simulink model "native_M10_payload5kg_pose_hold_r2"  (R2026b)
settings: Solver=ode4  StopTime=35  FixedStep=2.5e-05  MaxStep=0.001  RelTol=1e-5
InitFcn:
  | addpath(fileparts(get_param(bdroot,'FileName')));
values from neighbouring files (symbols this model uses):
  s = block.Dwork(1).Data    [native_M10_payload5kg_pose_hold_r2_controller.m]
undefined symbols (not defined in the file or in its folder): X, Y, Z
libraries: sm_lib x42, nesl_utility x20
(part 1 of 2)
settings Model: Creator=lelfs  LastModifiedBy=lelfs
settings DataIOCC: LimitDataPoints=on  MaxDataPoints=10000
settings OptimizationCC: LifeSpan=inf  ReuseModelBlockBuffer=off
settings DebuggingCC: AllowSymbolicDim=off  ArithmeticOperatorsInVariantConditions=warning  SFExecutionAtInitializationDiag=none  SFNoUnconditionalDefaultTransitionDiag=warning  SFUnexpectedBacktrackingDiag=warning  SubsystemReferenceDiagnosticForUnitTest=warning
settings SFSimCC: CustomCodeUndefinedFunction=UseInterfaceOnly  SimUseLocalCustomCode=off
settings RTWCC: DLArmComputeVersion=19.05  RTWUseLocalCustomCode=off
settings CodeAppCC: StateflowObjectComments=on
settings GRTTargetCC: TargetLangStandard=C89/C90 (ANSI)
settings ConfigComp: CovExternalEMLEnable=off  CovSFcnEnable=off  CovSaveCumulativeToWorkspaceVar=on  CovSaveSingleToWorkspaceVar=on
settings SimscapeCC: SimscapeLogLimitData=off  SimscapeUseEnergyAccounting=off
settings ExplorerConfigSet: SimMechanicsOpenEditorOnUpdate=off

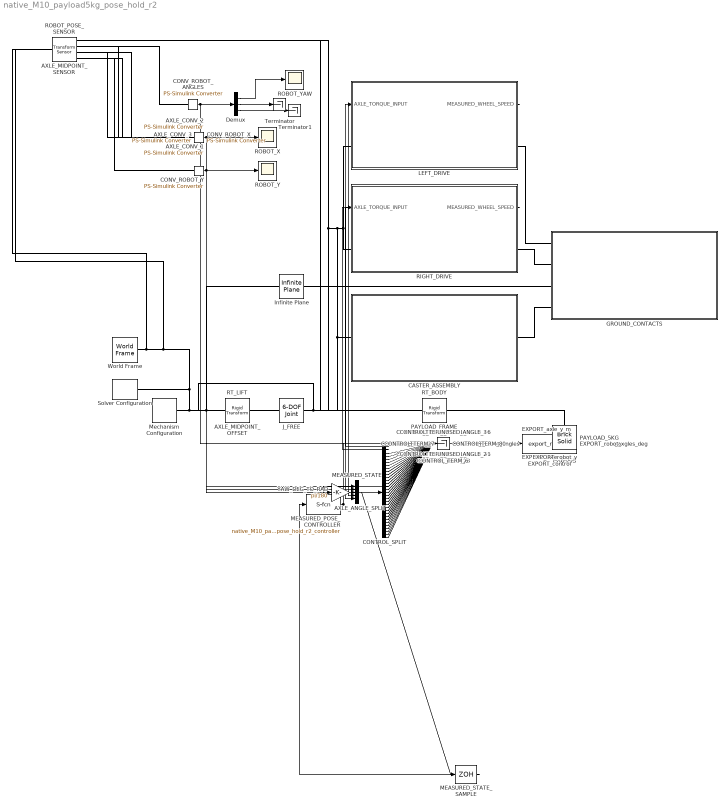
== system native_M10_payload5kg_pose_hold_r2 ==
  AXLE_ANGLE_SPLIT : Demux  Outputs=3
  AXLE_CONV_1 : nesl_utility/PS-Simulink Converter  PhysicalDomain=network_engine_domain  SubClassName=ps_output  LeftPortType=input  RightPortType=output  PseudoPeriodic=off  Frequencies=[]  VectorFormat=inherit  Unit=m  AffineConversion=off
  AXLE_CONV_2 : nesl_utility/PS-Simulink Converter  PhysicalDomain=network_engine_domain  SubClassName=ps_output  LeftPortType=input  RightPortType=output  PseudoPeriodic=off  Frequencies=[]  VectorFormat=inherit  Unit=m  AffineConversion=off
  AXLE_CONV_3 : nesl_utility/PS-Simulink Converter  PhysicalDomain=network_engine_domain  SubClassName=ps_output  LeftPortType=input  RightPortType=output  PseudoPeriodic=off  Frequencies=[]  VectorFormat=inherit  Unit=deg  AffineConversion=off
  AXLE_MIDPOINT_OFFSET : sm_lib/Frames and Transforms/Rigid Transform  RotationMethod=None  FollAlignAxisA=+X  BaseAlignAxisA=+Y  FollAlignAxisB=+Y  BaseAlignAxisB=+Z  RotationStandardAxis=+Z  RotationAngle=0  RotationAngleUnits=deg  RotationArbitraryAxis=[0 0 1]  RotationSequenceAxes=FollowerAxes  RotationSequence=XYX  RotationSequenceAngles=[0 0 0]  RotationSequenceAnglesUnits=deg  RotationMatrix=[1 0 0;0 1 0;0 0 1]  Quaternion=[1 0 0 0]  TranslationMethod=Cartesian  TranslationCartesianOffset=[0 0 0.075]  TranslationCartesianOffsetUnits=m  TranslationStandardAxis=+Z  TranslationStandardOffset=0  TranslationStandardOffsetUnits=m  TranslationROffset=0  TranslationROffsetUnits=m  TranslationThetaOffset=0  TranslationThetaOffsetUnits=deg  TranslationZOffset=0  TranslationZOffsetUnits=m
  AXLE_MIDPOINT_SENSOR : sm_lib/Frames and Transforms/Transform Sensor  ObservationFrame=World  ExpressedInFrame=World  RotationSequence=ZYX  SenseAngle=off  SenseAxis=off  SenseQ=off  SenseR=off  SenseRotationSequence=on  SenseOmegaX=off  SenseOmegaY=off  SenseOmegaZ=off  SenseOmega=off  SenseQDot=off  SenseRDot=off  SenseRotationSequenceDot=off  SenseAlphaX=off  SenseAlphaY=off  SenseAlphaZ=off  SenseAlpha=off  SenseQDDot=off  SenseRDDot=off  SenseX=on  SenseY=on  SenseZ=off  SenseXYZ=off  SenseRad=off  SenseAzim=off  SenseDist=off  SenseInc=off  SenseXDot=off  SenseYDot=off  SenseZDot=off  SenseXYZDot=off  SenseRadDot=off  SenseAzimDot=off  SenseDistDot=off  SenseIncDot=off  SenseXDDot=off  SenseYDDot=off  SenseZDDot=off  SenseXYZDDot=off  SenseRadDDot=off  SenseAzimDDot=off  SenseDistDDot=off  SenseIncDDot=off
  CASTER_ASSEMBLY : Subsystem
  CHASSIS : sm_lib/Body Elements/Brick Solid  BrickDimensions=[0.50 0.32 0.08]  BrickDimensionsUnits=m  ExportEntireGeometry=off  InertiaType=CalculateFromGeometry  BasedOnType=Mass  Density=1000  DensityUnits=kg/m^3  Mass=15.2  MassUnits=kg  CenterOfMass=[0 0 0]  CenterOfMassUnits=m  MomentsOfInertia=[1 1 1]  MomentsOfInertiaUnits=kg*m^2  ProductsOfInertia=[0 0 0]  ProductsOfInertiaUnits=kg*m^2  GraphicType=FromGeometry  MarkerShape=Sphere  MarkerSize=10  GraphicVisPropType=SimpleVisualProperties  GraphicDiffuseColor=[0.5 0.5 0.5]  GraphicOpacity=1.0  GraphicSpecularColor=[0.5 0.5 0.5 1.0]  GraphicAmbientColor=[0.15 0.15 0.15 1.0]  GraphicEmissiveColor=[0.0 0.0 0.0 1.0]  GraphicShininess=75  DoExposeReferenceFrame=on  SerializedFrames=<Frames/>
  CONTROL_SPLIT : Demux  Outputs=31
  CONTROL_TERM_{3..31} (29 alike) : Terminator
  CONV_ROBOT_ANGLES : nesl_utility/PS-Simulink Converter  PhysicalDomain=network_engine_domain  SubClassName=ps_output  LeftPortType=input  RightPortType=output  PseudoPeriodic=off  Frequencies=[]  VectorFormat=inherit  Unit=deg  AffineConversion=off
  CONV_ROBOT_X : nesl_utility/PS-Simulink Converter  PhysicalDomain=network_engine_domain  SubClassName=ps_output  LeftPortType=input  RightPortType=output  PseudoPeriodic=off  Frequencies=[]  VectorFormat=inherit  Unit=m  AffineConversion=off
  CONV_ROBOT_Y : nesl_utility/PS-Simulink Converter  PhysicalDomain=network_engine_domain  SubClassName=ps_output  LeftPortType=input  RightPortType=output  PseudoPeriodic=off  Frequencies=[]  VectorFormat=inherit  Unit=m  AffineConversion=off
  Demux : Demux  Outputs=3
  EXPORT_axle_angles_deg : ToWorkspace  VariableName=export_axle_angles_deg  SaveFormat=Timeseries  SampleTime=0.001
  EXPORT_axle_x_m : ToWorkspace  VariableName=export_axle_x_m  SaveFormat=Timeseries  SampleTime=0.001
  EXPORT_axle_y_m : ToWorkspace  VariableName=export_axle_y_m  SaveFormat=Timeseries  SampleTime=0.001
  EXPORT_control : ToWorkspace  VariableName=export_control  SaveFormat=Timeseries  SampleTime=0.001
  EXPORT_robot_angles : ToWorkspace  VariableName=export_robot_angles  SaveFormat=Timeseries  SampleTime=0.001
  EXPORT_robot_x : ToWorkspace  VariableName=export_robot_x  SaveFormat=Timeseries  SampleTime=0.001
  EXPORT_robot_y : ToWorkspace  VariableName=export_robot_y  SaveFormat=Timeseries  SampleTime=0.001
  GROUND_CONTACTS : Subsystem
  Infinite Plane : sm_lib/Curves and Surfaces/Infinite Plane  GraphicType=Rectangle  GraphicPlaneWidth=3  GraphicPlaneWidthUnits=m  GraphicPlaneHeight=3  GraphicPlaneHeightUnits=m  GraphicVisPropType=SimpleVisualProperties  GraphicDiffuseColor=[0.5 0.5 0.5]  GraphicOpacity=1  GraphicSpecularColor=[0.5 0.5 0.5 1.0]  GraphicAmbientColor=[0.15 0.15 0.15 1.0]  GraphicEmissiveColor=[0.0 0.0 0.0 1.0]  GraphicShininess=75
  J_FREE : sm_lib/Joints/6-DOF Joint  JointMode=Normal  CompositeWrenchDir=FollowerOnBase  CompositeWrenchFrame=BaseFrame  SenseConstraintForce=off  SenseConstraintTorque=off  SenseTotalForce=off  SenseTotalTorque=off  PxPositionTargetSpecify=on  PxPositionTargetPriority=High  PxPositionTargetValue=0  PxPositionTargetValueUnits=m  PxVelocityTargetSpecify=on  PxVelocityTargetPriority=High  PxVelocityTargetValue=0  PxVelocityTargetValueUnits=m/s  PxEquilibriumPosition=0  PxEquilibriumPositionUnits=m  PxSpringStiffness=0  PxSpringStiffnessUnits=N/m  PxDampingCoefficient=0  PxDampingCoefficientUnits=N/(m/s)  PxLowerLimitSpecify=off  PxLowerLimitBound=-1  PxLowerLimitBoundUnits=m  PxLowerLimitStiffness=1e6  PxLowerLimitStiffnessUnits=N/m  PxLowerLimitDamping=1e3  PxLowerLimitDampingUnits=N/(m/s)  PxLowerLimitTransitionRegionWidth=1e-4  PxLowerLimitTransitionRegionWidthUnits=m  PxUpperLimitSpecify=off  PxUpperLimitBound=1  PxUpperLimitBoundUnits=m  PxUpperLimitStiffness=1e6  PxUpperLimitStiffnessUnits=N/m  PxUpperLimitDamping=1e3  PxUpperLimitDampingUnits=N/(m/s)  PxUpperLimitTransitionRegionWidth=1e-4  PxUpperLimitTransitionRegionWidthUnits=m  PxTorqueActuationMode=NoTorque  PxMotionActuationMode=ComputedMotion  PxSensePosition=off  PxSenseVelocity=off  PxSenseAcceleration=off  PxSenseTorqueForce=off  PxSenseLowerLimitTorqueForce=off  PxSenseUpperLimitTorqueForce=off  PyPositionTargetSpecify=on  PyPositionTargetPriority=High  PyPositionTargetValue=0  PyPositionTargetValueUnits=m  PyVelocityTargetSpecify=on  PyVelocityTargetPriority=High  PyVelocityTargetValue=0  PyVelocityTargetValueUnits=m/s  PyEquilibriumPosition=0  PyEquilibriumPositionUnits=m  PySpringStiffness=0  PySpringStiffnessUnits=N/m  PyDampingCoefficient=0  PyDampingCoefficientUnits=N/(m/s)  PyLowerLimitSpecify=off  PyLowerLimitBound=-1  PyLowerLimitBoundUnits=m  PyLowerLimitStiffness=1e6  PyLowerLimitStiffnessUnits=N/m  PyLowerLimitDamping=1e3  PyLowerLimitDampingUnits=N/(m/s)  PyLowerLimitTransitionRegionWidth=1e-4  PyLowerLimitTransitionRegionWidthUnits=m  PyUpperLimitSpecify=off  PyUpperLimitBound=1  PyUpperLimitBoundUnits=m  PyUpperLimitStiffness=1e6  PyUpperLimitStiffnessUnits=N/m  PyUpperLimitDamping=1e3  PyUpperLimitDampingUnits=N/(m/s)  PyUpperLimitTransitionRegionWidth=1e-4  PyUpperLimitTransitionRegionWidthUnits=m  PyTorqueActuationMode=NoTorque  PyMotionActuationMode=ComputedMotion  PySensePosition=off  PySenseVelocity=off  PySenseAcceleration=off  PySenseTorqueForce=off  PySenseLowerLimitTorqueForce=off  PySenseUpperLimitTorqueForce=off  PzPositionTargetSpecify=on  PzPositionTargetPriority=High  PzPositionTargetValue=0  PzPositionTargetValueUnits=m  PzVelocityTargetSpecify=on  PzVelocityTargetPriority=High  PzVelocityTargetValue=0  PzVelocityTargetValueUnits=m/s  PzEquilibriumPosition=0  PzEquilibriumPositionUnits=m  PzSpringStiffness=0  PzSpringStiffnessUnits=N/m  PzDampingCoefficient=0  PzDampingCoefficientUnits=N/(m/s)  PzLowerLimitSpecify=off  PzLowerLimitBound=-1  PzLowerLimitBoundUnits=m  PzLowerLimitStiffness=1e6  PzLowerLimitStiffnessUnits=N/m  PzLowerLimitDamping=1e3  PzLowerLimitDampingUnits=N/(m/s)  PzLowerLimitTransitionRegionWidth=1e-4  PzLowerLimitTransitionRegionWidthUnits=m  PzUpperLimitSpecify=off  PzUpperLimitBound=1  PzUpperLimitBoundUnits=m  PzUpperLimitStiffness=1e6  PzUpperLimitStiffnessUnits=N/m  PzUpperLimitDamping=1e3  PzUpperLimitDampingUnits=N/(m/s)  PzUpperLimitTransitionRegionWidth=1e-4  PzUpperLimitTransitionRegionWidthUnits=m  PzTorqueActuationMode=NoTorque  PzMotionActuationMode=ComputedMotion  PzSensePosition=off  PzSenseVelocity=off  PzSenseAcceleration=off  PzSenseTorqueForce=off  PzSenseLowerLimitTorqueForce=off  PzSenseUpperLimitTorqueForce=off  SphPositionTargetSpecify=on  SphPositionTargetPriority=High  SphPositionTargetRotationMethod=None  SphPositionTargetFollAlignAxisA=+X  SphPositionTargetBaseAlignAxisA=+Y  SphPositionTargetFollAlignAxisB=+Y  SphPositionTargetBaseAlignAxisB=+Z  SphPositionTargetRotationStandardAxis=+Z  SphPositionTargetRotationAngle=0  SphPositionTargetRotationAngleUnits=deg  SphPositionTargetRotationArbitraryAxis=[0 0 1]  SphPositionTargetRotationSequenceAxes=FollowerAxes  SphPositionTargetRotationSequence=XYX  SphPositionTargetRotationSequenceAngles=[0 0 0]  SphPositionTargetRotationSequenceAnglesUnits=deg  SphPositionTargetRotationMatrix=[1 0 0;0 1 0;0 0 1]  SphPositionTargetQuaternion=[1 0 0 0]  SphVelocityTargetSpecify=on  SphVelocityTargetPriority=High  SphVelocityTargetValue=[0 0 0]  SphVelocityTargetValueUnits=rad/s  SphVelocityTargetInFollowerFrame=on  SphEqPosRotationMethod=None  SphEqPosFollAlignAxisA=+X  SphEqPosBaseAlignAxisA=+Y  SphEqPosFollAlignAxisB=+Y  SphEqPosBaseAlignAxisB=+Z  SphEqPosRotationStandardAxis=+Z  SphEqPosRotationAngle=0  SphEqPosRotationAngleUnits=deg  SphEqPosRotationArbitraryAxis=[0 0 1]  SphEqPosRotationSequenceAxes=FollowerAxes  SphEqPosRotationSequence=XYX  SphEqPosRotationSequenceAngles=[0 0 0]  SphEqPosRotationSequenceAnglesUnits=deg  SphEqPosRotationMatrix=[1 0 0;0 1 0;0 0 1]  SphEqPosQuaternion=[1 0 0 0]  SphSpringStiffness=0  SphSpringStiffnessUnits=N*m/deg  SphDampingCoefficient=0  SphDampingCoefficientUnits=N*m/(deg/s)  SphLowerLimitSpecify=off  SphLowerLimitBound=15  SphLowerLimitBoundUnits=deg  SphLowerLimitStiffness=1e4  SphLowerLimitStiffnessUnits=N*m/deg  SphLowerLimitDamping=10  SphLowerLimitDampingUnits=N*m/(deg/s)  SphLowerLimitTransitionRegionWidth=0.1  SphLowerLimitTransitionRegionWidthUnits=deg  SphUpperLimitSpecify=off  SphUpperLimitBound=45  SphUpperLimitBoundUnits=deg  SphUpperLimitStiffness=1e4  SphUpperLimitStiffnessUnits=N*m/deg  SphUpperLimitDamping=10  SphUpperLimitDampingUnits=N*m/(deg/s)  SphUpperLimitTransitionRegionWidth=0.1  SphUpperLimitTransitionRegionWidthUnits=deg  SphTorqueActuationMode=NoTorque  SphActuateTorqueX=off  SphActuateTorqueY=off  SphActuateTorqueZ=off  SphActuateTorque=off  SphActuationFrame=BaseFrame  SphSensePosition=off  SphSenseVelocityX=off  SphSenseVelocityY=off  SphSenseVelocityZ=off  SphSenseVelocity=off  SphSenseAccelerationX=off  SphSenseAccelerationY=off  SphSenseAccelerationZ=off  SphSenseAcceleration=off  SphSenseLowerLimitTorqueMag=off  SphSenseUpperLimitTorqueMag=off  SphSensingFrame=BaseFrame
  LEFT_DRIVE : Subsystem
  MEASURED_POSE_CONTROLLER : M-S-Function  FunctionName=native_M10_payload5kg_pose_hold_r2_controller  Parameters=110
  MEASURED_STATE : Mux  Inputs=5
  MEASURED_STATE_SAMPLE : ZeroOrderHold  SampleTime=.01
  Mechanism Configuration : sm_lib/Utilities/Mechanism Configuration  UniformGravity=Constant  GravityVector=[0 0 -9.81]  GravityVectorUnits=m/s^2  LinearizationDelta=0.001  JointModeTransitionNonlinearIterations=2
  PAYLOAD_5KG : sm_lib/Body Elements/Brick Solid  BrickDimensions=[.2 .2 .15]  BrickDimensionsUnits=m  ExportEntireGeometry=off  InertiaType=CalculateFromGeometry  BasedOnType=Mass  Density=1000  DensityUnits=kg/m^3  Mass=5  MassUnits=kg  CenterOfMass=[0 0 0]  CenterOfMassUnits=m  MomentsOfInertia=[1 1 1]  MomentsOfInertiaUnits=kg*m^2  ProductsOfInertia=[0 0 0]  ProductsOfInertiaUnits=kg*m^2  GraphicType=FromGeometry  MarkerShape=Sphere  MarkerSize=10  GraphicVisPropType=SimpleVisualProperties  GraphicDiffuseColor=[0.5 0.5 0.5]  GraphicOpacity=1.0  GraphicSpecularColor=[0.5 0.5 0.5 1.0]  GraphicAmbientColor=[0.15 0.15 0.15 1.0]  GraphicEmissiveColor=[0.0 0.0 0.0 1.0]  GraphicShininess=75  DoExposeReferenceFrame=on  SerializedFrames=<Frames/>
  PAYLOAD_FRAME : sm_lib/Frames and Transforms/Rigid Transform  RotationMethod=None  FollAlignAxisA=+X  BaseAlignAxisA=+Y  FollAlignAxisB=+Y  BaseAlignAxisB=+Z  RotationStandardAxis=+Z  RotationAngle=0.0  RotationAngleUnits=deg  RotationArbitraryAxis=[0 0 1]  RotationSequenceAxes=FollowerAxes  RotationSequence=XYX  RotationSequenceAngles=[0 0 0]  RotationSequenceAnglesUnits=deg  RotationMatrix=[1 0 0; 0 1 0; 0 0 1]  Quaternion=[1 0 0 0]  TranslationMethod=Cartesian  TranslationCartesianOffset=[-.04 0 .23]  TranslationCartesianOffsetUnits=m  TranslationStandardAxis=+Z  TranslationStandardOffset=0  TranslationStandardOffsetUnits=m  TranslationROffset=0  TranslationROffsetUnits=m  TranslationThetaOffset=0  TranslationThetaOffsetUnits=deg  TranslationZOffset=0  TranslationZOffsetUnits=m
  RIGHT_DRIVE : Subsystem
  ROBOT_POSE_SENSOR : sm_lib/Frames and Transforms/Transform Sensor  ObservationFrame=World  ExpressedInFrame=World  RotationSequence=ZYX  SenseAngle=off  SenseAxis=off  SenseQ=off  SenseR=off  SenseRotationSequence=on  SenseOmegaX=off  SenseOmegaY=off  SenseOmegaZ=off  SenseOmega=off  SenseQDot=off  SenseRDot=off  SenseRotationSequenceDot=off  SenseAlphaX=off  SenseAlphaY=off  SenseAlphaZ=off  SenseAlpha=off  SenseQDDot=off  SenseRDDot=off  SenseX=on  SenseY=on  SenseZ=off  SenseXYZ=off  SenseRad=off  SenseAzim=off  SenseDist=off  SenseInc=off  SenseXDot=off  SenseYDot=off  SenseZDot=off  SenseXYZDot=off  SenseRadDot=off  SenseAzimDot=off  SenseDistDot=off  SenseIncDot=off  SenseXDDot=off  SenseYDDot=off  SenseZDDot=off  SenseXYZDDot=off  SenseRadDDot=off  SenseAzimDDot=off  SenseDistDDot=off  SenseIncDDot=off
  ROBOT_X : Scope
      settings: ActiveDisplayYMinimum=0.0098960856448418733  ActiveDisplayYMaximum=0.010138629193924146  DataLoggingVariableName=ScopeData6
  ROBOT_Y : Scope
      settings: ActiveDisplayYMinimum=-3.9078256415425135E-8  ActiveDisplayYMaximum=3.95768930877411E-8  DataLoggingVariableName=ScopeData7
  ROBOT_YAW : Scope
      settings: ActiveDisplayYMinimum=-1.503968067414708E-5  ActiveDisplayYMaximum=1.0251655988243249E-5  DataLoggingVariableName=ScopeData8
  RT_BODY : sm_lib/Frames and Transforms/Rigid Transform  RotationMethod=None  FollAlignAxisA=+X  BaseAlignAxisA=+Y  FollAlignAxisB=+Y  BaseAlignAxisB=+Z  RotationStandardAxis=+Z  RotationAngle=0.0  RotationAngleUnits=deg  RotationArbitraryAxis=[0 0 1]  RotationSequenceAxes=FollowerAxes  RotationSequence=XYX  RotationSequenceAngles=[0 0 0]  RotationSequenceAnglesUnits=deg  RotationMatrix=[1 0 0; 0 1 0; 0 0 1]  Quaternion=[1 0 0 0]  TranslationMethod=Cartesian  TranslationCartesianOffset=[-0.084210526 0 0.122368421]  TranslationCartesianOffsetUnits=m  TranslationStandardAxis=+Z  TranslationStandardOffset=0  TranslationStandardOffsetUnits=m  TranslationROffset=0  TranslationROffsetUnits=m  TranslationThetaOffset=0  TranslationThetaOffsetUnits=deg  TranslationZOffset=0  TranslationZOffsetUnits=m
  RT_LIFT : sm_lib/Frames and Transforms/Rigid Transform  RotationMethod=None  FollAlignAxisA=+X  BaseAlignAxisA=+Y  FollAlignAxisB=+Y  BaseAlignAxisB=+Z  RotationStandardAxis=+Z  RotationAngle=0  RotationAngleUnits=deg  RotationArbitraryAxis=[0 0 1]  RotationSequenceAxes=FollowerAxes  RotationSequence=XYX  RotationSequenceAngles=[0 0 0]  RotationSequenceAnglesUnits=deg  RotationMatrix=[1 0 0;0 1 0;0 0 1]  Quaternion=[1 0 0 0]  TranslationMethod=Cartesian  TranslationCartesianOffset=[0 0 0.005]  TranslationCartesianOffsetUnits=m  TranslationStandardAxis=+Z  TranslationStandardOffset=0  TranslationStandardOffsetUnits=m  TranslationROffset=0  TranslationROffsetUnits=m  TranslationThetaOffset=0  TranslationThetaOffsetUnits=deg  TranslationZOffset=0  TranslationZOffsetUnits=m
  Solver Configuration : nesl_utility/Solver Configuration  PhysicalDomain=network_engine_domain  SubClassName=solver  LeftPortType=input  RightPortType=generic  Tones=[]  Harmonics=[]  SimulateNoise=off  Profile=off  UseLocalSampling=off  EnableSwitchedLinearOptims=on  FrequencyDomain=off  UseCCode=off  RelTol=0.001  AbsTol=1e-06  MinStep=1e-09  ToWorkspace=off  RevertToSquareIcSolve=off  NumHomotopyIterations=100  PhasorMode=off  PhasorModeNumHarmonics=1  ConsistencySolver=NEWTON_XTOL_AFTER_FTOL  CanonicalOrdering=UNORDERED  OptimizeIntermediates=UNOPTIMIZED  MulticoreSolverChoice=BACKWARD_EULER  IndexReductionMethod=DerivativeReplacement  DoDC=off  ResidualTolerance=1e-09  ConsistencyTolSource=GLOBAL  ConsistencyAbsTol=0.001  ConsistencyRelTol=0.001  ConsistencyTolFactor=0.001  UseLocalSolver=off  LocalSolverChoice=NE_BACKWARD_EULER_ADVANCER  ResolveIndetEquations=on  FunctionEvalNumThread=1  LocalSolverSampleTime=0.001  DoFixedCost=off  MaxNonlinIter=3  MaxModeIter=2  ComputeImpulses=off  ImpulseIterations=2  LinearAlgebra=Sparse  LinearAlgebraNumThread=0  EquationFormulation=NE_TIME_EF  DelaysMemoryBudget=1024  AutomaticFiltering=on  FilteringTimeConstant=0.001  PartitionStorageMethod=AS_NEEDED  PartitionMemoryBudget=1024  PartitionMethod=FAST  MultibodyUseLocalSolver=off  MultibodyLocalSolverChoice=ODE1  MultibodyLocalSolverSampleTime=0.001
  Terminator : Terminator
  Terminator1 : Terminator
  UNUSED_ANGLE_2 : Terminator
  UNUSED_ANGLE_3 : Terminator
  World Frame : sm_lib/Frames and Transforms/World Frame
  YAW_DEG_TO_RAD : Gain  Gain=pi/180
  wires:
  CONV_ROBOT_X/1 -> ROBOT_X/1, EXPORT_robot_x/1
  CONV_ROBOT_Y/1 -> ROBOT_Y/1, EXPORT_robot_y/1
  CONV_ROBOT_ANGLES/1 -> Demux/1, EXPORT_robot_angles/1
  Demux/3 -> Terminator1/1
  Demux/2 -> Terminator/1
  Demux/1 -> ROBOT_YAW/1
  AXLE_CONV_1/1 -> EXPORT_axle_x_m/1, MEASURED_STATE/1
  AXLE_CONV_2/1 -> EXPORT_axle_y_m/1, MEASURED_STATE/2
  AXLE_CONV_3/1 -> EXPORT_axle_angles_deg/1, AXLE_ANGLE_SPLIT/1
  AXLE_ANGLE_SPLIT/1 -> YAW_DEG_TO_RAD/1
  AXLE_ANGLE_SPLIT/2 -> UNUSED_ANGLE_2/1
  AXLE_ANGLE_SPLIT/3 -> UNUSED_ANGLE_3/1
  YAW_DEG_TO_RAD/1 -> MEASURED_STATE/3
  LEFT_DRIVE/1(MEASURED_WHEEL_SPEED) -> MEASURED_STATE/4
  RIGHT_DRIVE/1(MEASURED_WHEEL_SPEED) -> MEASURED_STATE/5
  MEASURED_STATE/1 -> MEASURED_STATE_SAMPLE/1
  MEASURED_STATE_SAMPLE/1 -> MEASURED_POSE_CONTROLLER/1
  MEASURED_POSE_CONTROLLER/1 -> CONTROL_SPLIT/1, EXPORT_control/1
  CONTROL_SPLIT/1 -> LEFT_DRIVE/1(AXLE_TORQUE_INPUT)
  CONTROL_SPLIT/2 -> RIGHT_DRIVE/1(AXLE_TORQUE_INPUT)
  CONTROL_SPLIT/3 -> CONTROL_TERM_3/1
  CONTROL_SPLIT/4 -> CONTROL_TERM_4/1
  CONTROL_SPLIT/5 -> CONTROL_TERM_5/1
  CONTROL_SPLIT/6 -> CONTROL_TERM_6/1
  CONTROL_SPLIT/7 -> CONTROL_TERM_7/1
  CONTROL_SPLIT/8 -> CONTROL_TERM_8/1
  CONTROL_SPLIT/9 -> CONTROL_TERM_9/1
  CONTROL_SPLIT/10 -> CONTROL_TERM_10/1
  CONTROL_SPLIT/11 -> CONTROL_TERM_11/1
  CONTROL_SPLIT/12 -> CONTROL_TERM_12/1
  CONTROL_SPLIT/13 -> CONTROL_TERM_13/1
  CONTROL_SPLIT/14 -> CONTROL_TERM_14/1
  CONTROL_SPLIT/15 -> CONTROL_TERM_15/1
  CONTROL_SPLIT/16 -> CONTROL_TERM_16/1
  CONTROL_SPLIT/17 -> CONTROL_TERM_17/1
  CONTROL_SPLIT/18 -> CONTROL_TERM_18/1
  CONTROL_SPLIT/19 -> CONTROL_TERM_19/1
  CONTROL_SPLIT/20 -> CONTROL_TERM_20/1
  CONTROL_SPLIT/21 -> CONTROL_TERM_21/1
  CONTROL_SPLIT/22 -> CONTROL_TERM_22/1
  CONTROL_SPLIT/23 -> CONTROL_TERM_23/1
  CONTROL_SPLIT/24 -> CONTROL_TERM_24/1
  CONTROL_SPLIT/25 -> CONTROL_TERM_25/1
  CONTROL_SPLIT/26 -> CONTROL_TERM_26/1
  CONTROL_SPLIT/27 -> CONTROL_TERM_27/1
  CONTROL_SPLIT/28 -> CONTROL_TERM_28/1
  CONTROL_SPLIT/29 -> CONTROL_TERM_29/1
  CONTROL_SPLIT/30 -> CONTROL_TERM_30/1
  CONTROL_SPLIT/31 -> CONTROL_TERM_31/1
  connections:
  RIGHT_DRIVE/RConn1 -- GROUND_CONTACTS/LConn2
  Mechanism Configuration/RConn1 -- Infinite Plane/LConn1 -- RT_LIFT/LConn1 -- ROBOT_POSE_SENSOR/LConn1 -- World Frame/RConn1 -- AXLE_MIDPOINT_SENSOR/LConn1 -- Solver Configuration/RConn1
  RT_BODY/RConn1 -- CHASSIS/RConn1
  RT_LIFT/RConn1 -- J_FREE/LConn1
  LEFT_DRIVE/RConn1 -- GROUND_CONTACTS/LConn1
  J_FREE/RConn1 -- AXLE_MIDPOINT_OFFSET/LConn1 -- PAYLOAD_FRAME/LConn1 -- ROBOT_POSE_SENSOR/RConn1 -- CASTER_ASSEMBLY/LConn1 -- RT_BODY/LConn1 -- LEFT_DRIVE/LConn1 -- RIGHT_DRIVE/LConn1
  Infinite Plane/RConn1 -- GROUND_CONTACTS/LConn3
  CASTER_ASSEMBLY/RConn1 -- GROUND_CONTACTS/LConn4
  CONV_ROBOT_X/LConn1 -- ROBOT_POSE_SENSOR/RConn3
  ROBOT_POSE_SENSOR/RConn4 -- CONV_ROBOT_Y/LConn1
  ROBOT_POSE_SENSOR/RConn2 -- CONV_ROBOT_ANGLES/LConn1
  AXLE_MIDPOINT_OFFSET/RConn1 -- AXLE_MIDPOINT_SENSOR/RConn1
  AXLE_MIDPOINT_SENSOR/RConn3 -- AXLE_CONV_1/LConn1
  AXLE_MIDPOINT_SENSOR/RConn4 -- AXLE_CONV_2/LConn1
  AXLE_MIDPOINT_SENSOR/RConn2 -- AXLE_CONV_3/LConn1
  PAYLOAD_FRAME/RConn1 -- PAYLOAD_5KG/RConn1

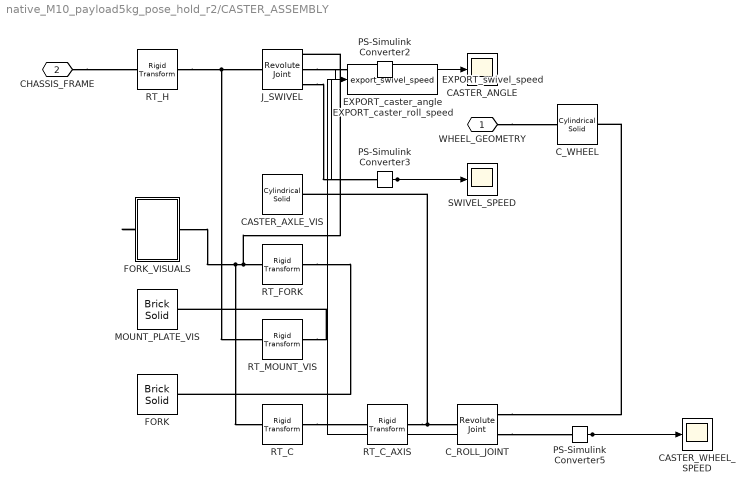
== system native_M10_payload5kg_pose_hold_r2/CASTER_ASSEMBLY ==
  CASTER_ANGLE : Scope
      settings: ActiveDisplayYMinimum=-1.4905941887815928  ActiveDisplayYMaximum=1.2443135814952986  DataLoggingMaxPoints=2000  DataLoggingVariableName=ScopeData2
  CASTER_AXLE_VIS : sm_lib/Body Elements/Cylindrical Solid  CylinderRadius=0.004  CylinderRadiusUnits=m  CylinderLength=0.040  CylinderLengthUnits=m  ExportEntireGeometry=off  InertiaType=Custom  BasedOnType=Density  Density=1000  DensityUnits=kg/m^3  Mass=0  MassUnits=kg  CenterOfMass=[0 0 0]  CenterOfMassUnits=m  MomentsOfInertia=[0 0 0]  MomentsOfInertiaUnits=kg*m^2  ProductsOfInertia=[0 0 0]  ProductsOfInertiaUnits=kg*m^2  GraphicType=FromGeometry  MarkerShape=Sphere  MarkerSize=10  GraphicVisPropType=SimpleVisualProperties  GraphicDiffuseColor=[0.75 0.77 0.80]  GraphicOpacity=1  GraphicSpecularColor=[0.5 0.5 0.5 1.0]  GraphicAmbientColor=[0.15 0.15 0.15 1.0]  GraphicEmissiveColor=[0.0 0.0 0.0 1.0]  GraphicShininess=75  DoExposeReferenceFrame=on  SerializedFrames=<Frames/>
  CASTER_WHEEL_SPEED : Scope
      settings: ActiveDisplayYMinimum=0.88573921875000006  ActiveDisplayYMaximum=1.1288404687500002  DataLoggingMaxPoints=2000  DataLoggingVariableName=ScopeData4
  C_ROLL_JOINT : sm_lib/Joints/Revolute Joint  JointMode=Normal  CompositeWrenchDir=FollowerOnBase  CompositeWrenchFrame=BaseFrame  SenseConstraintForce=off  SenseConstraintTorque=off  SenseTotalForce=off  SenseTotalTorque=off  PositionTargetSpecify=on  PositionTargetPriority=High  PositionTargetValue=0  PositionTargetValueUnits=deg  VelocityTargetSpecify=on  VelocityTargetPriority=High  VelocityTargetValue=0  VelocityTargetValueUnits=rad/s  EquilibriumPosition=0  EquilibriumPositionUnits=deg  SpringStiffness=0  SpringStiffnessUnits=N*m/deg  DampingCoefficient=0  DampingCoefficientUnits=N*m/(deg/s)  LowerLimitSpecify=off  LowerLimitBound=-90  LowerLimitBoundUnits=deg  LowerLimitStiffness=1e4  LowerLimitStiffnessUnits=N*m/deg  LowerLimitDamping=10  LowerLimitDampingUnits=N*m/(deg/s)  LowerLimitTransitionRegionWidth=0.1  LowerLimitTransitionRegionWidthUnits=deg  UpperLimitSpecify=off  UpperLimitBound=90  UpperLimitBoundUnits=deg  UpperLimitStiffness=1e4  UpperLimitStiffnessUnits=N*m/deg  UpperLimitDamping=10  UpperLimitDampingUnits=N*m/(deg/s)  UpperLimitTransitionRegionWidth=0.1  UpperLimitTransitionRegionWidthUnits=deg  TorqueActuationMode=NoTorque  MotionActuationMode=ComputedMotion  SensePosition=off  SenseVelocity=on  SenseAcceleration=off  SenseTorqueForce=off  SenseLowerLimitTorqueForce=off  SenseUpperLimitTorqueForce=off
  C_WHEEL : sm_lib/Body Elements/Cylindrical Solid  CylinderRadius=0.04  CylinderRadiusUnits=m  CylinderLength=0.02  CylinderLengthUnits=m  ExportEntireGeometry=on  InertiaType=CalculateFromGeometry  BasedOnType=Mass  Density=1000  DensityUnits=kg/m^3  Mass=0.4  MassUnits=kg  CenterOfMass=[0 0 0]  CenterOfMassUnits=m  MomentsOfInertia=[1 1 1]  MomentsOfInertiaUnits=kg*m^2  ProductsOfInertia=[0 0 0]  ProductsOfInertiaUnits=kg*m^2  GraphicType=FromGeometry  MarkerShape=Sphere  MarkerSize=10  GraphicVisPropType=SimpleVisualProperties  GraphicDiffuseColor=[0.5 0.5 0.5]  GraphicOpacity=1  GraphicSpecularColor=[0.5 0.5 0.5 1.0]  GraphicAmbientColor=[0.15 0.15 0.15 1.0]  GraphicEmissiveColor=[0.0 0.0 0.0 1.0]  GraphicShininess=75  DoExposeReferenceFrame=on  SerializedFrames=<Frames/>
  EXPORT_caster_angle : ToWorkspace  VariableName=export_caster_angle  SaveFormat=Timeseries  SampleTime=0.001
  EXPORT_caster_roll_speed : ToWorkspace  VariableName=export_caster_roll_speed  SaveFormat=Timeseries  SampleTime=0.001
  EXPORT_swivel_speed : ToWorkspace  VariableName=export_swivel_speed  SaveFormat=Timeseries  SampleTime=0.001
  FORK : sm_lib/Body Elements/Brick Solid  BrickDimensions=[0.05 0.026 0.006]  BrickDimensionsUnits=m  ExportEntireGeometry=off  InertiaType=CalculateFromGeometry  BasedOnType=Mass  Density=1000  DensityUnits=kg/m^3  Mass=0.2  MassUnits=kg  CenterOfMass=[0 0 0]  CenterOfMassUnits=m  MomentsOfInertia=[1 1 1]  MomentsOfInertiaUnits=kg*m^2  ProductsOfInertia=[0 0 0]  ProductsOfInertiaUnits=kg*m^2  GraphicType=None  MarkerShape=Sphere  MarkerSize=10  GraphicVisPropType=SimpleVisualProperties  GraphicDiffuseColor=[0.5 0.5 0.5]  GraphicOpacity=1  GraphicSpecularColor=[0.5 0.5 0.5 1.0]  GraphicAmbientColor=[0.15 0.15 0.15 1.0]  GraphicEmissiveColor=[0.0 0.0 0.0 1.0]  GraphicShininess=75  DoExposeReferenceFrame=on  SerializedFrames=<Frames/>
  FORK_VISUALS : Subsystem
  J_SWIVEL : sm_lib/Joints/Revolute Joint  JointMode=Normal  CompositeWrenchDir=FollowerOnBase  CompositeWrenchFrame=BaseFrame  SenseConstraintForce=off  SenseConstraintTorque=off  SenseTotalForce=off  SenseTotalTorque=off  PositionTargetSpecify=on  PositionTargetPriority=High  PositionTargetValue=0  PositionTargetValueUnits=deg  VelocityTargetSpecify=on  VelocityTargetPriority=High  VelocityTargetValue=0  VelocityTargetValueUnits=rad/s  EquilibriumPosition=0  EquilibriumPositionUnits=deg  SpringStiffness=0  SpringStiffnessUnits=N*m/deg  DampingCoefficient=0.004  DampingCoefficientUnits=N*m/(rad/s)  LowerLimitSpecify=off  LowerLimitBound=-90  LowerLimitBoundUnits=deg  LowerLimitStiffness=1e4  LowerLimitStiffnessUnits=N*m/deg  LowerLimitDamping=10  LowerLimitDampingUnits=N*m/(deg/s)  LowerLimitTransitionRegionWidth=0.1  LowerLimitTransitionRegionWidthUnits=deg  UpperLimitSpecify=off  UpperLimitBound=90  UpperLimitBoundUnits=deg  UpperLimitStiffness=1e4  UpperLimitStiffnessUnits=N*m/deg  UpperLimitDamping=10  UpperLimitDampingUnits=N*m/(deg/s)  UpperLimitTransitionRegionWidth=0.1  UpperLimitTransitionRegionWidthUnits=deg  TorqueActuationMode=NoTorque  MotionActuationMode=ComputedMotion  SensePosition=on  SenseVelocity=on  SenseAcceleration=off  SenseTorqueForce=off  SenseLowerLimitTorqueForce=off  SenseUpperLimitTorqueForce=off
  MOUNT_PLATE_VIS : sm_lib/Body Elements/Brick Solid  BrickDimensions=[0.04 0.04 0.006]  BrickDimensionsUnits=m  ExportEntireGeometry=off  InertiaType=Custom  BasedOnType=Mass  Density=1000  DensityUnits=kg/m^3  Mass=0  MassUnits=kg  CenterOfMass=[0 0 0]  CenterOfMassUnits=m  MomentsOfInertia=[0 0 0]  MomentsOfInertiaUnits=kg*m^2  ProductsOfInertia=[0 0 0]  ProductsOfInertiaUnits=kg*m^2  GraphicType=FromGeometry  MarkerShape=Sphere  MarkerSize=10  GraphicVisPropType=SimpleVisualProperties  GraphicDiffuseColor=[0.35 0.38 0.42]  GraphicOpacity=1  GraphicSpecularColor=[0.5 0.5 0.5 1.0]  GraphicAmbientColor=[0.15 0.15 0.15 1.0]  GraphicEmissiveColor=[0.0 0.0 0.0 1.0]  GraphicShininess=75  DoExposeReferenceFrame=on  SerializedFrames=<Frames/>
  PS-Simulink Converter2 : nesl_utility/PS-Simulink Converter  PhysicalDomain=network_engine_domain  SubClassName=ps_output  LeftPortType=input  RightPortType=output  PseudoPeriodic=off  Frequencies=[]  VectorFormat=inherit  Unit=deg  AffineConversion=off
  PS-Simulink Converter3 : nesl_utility/PS-Simulink Converter  PhysicalDomain=network_engine_domain  SubClassName=ps_output  LeftPortType=input  RightPortType=output  PseudoPeriodic=off  Frequencies=[]  VectorFormat=inherit  Unit=rad/s  AffineConversion=off
  PS-Simulink Converter5 : nesl_utility/PS-Simulink Converter  PhysicalDomain=network_engine_domain  SubClassName=ps_output  LeftPortType=input  RightPortType=output  PseudoPeriodic=off  Frequencies=[]  VectorFormat=inherit  Unit=rad/s  AffineConversion=off
  RT_C : sm_lib/Frames and Transforms/Rigid Transform  RotationMethod=None  FollAlignAxisA=+X  BaseAlignAxisA=+Y  FollAlignAxisB=+Y  BaseAlignAxisB=+Z  RotationStandardAxis=+Z  RotationAngle=0  RotationAngleUnits=deg  RotationArbitraryAxis=[0 0 1]  RotationSequenceAxes=FollowerAxes  RotationSequence=XYX  RotationSequenceAngles=[0 0 0]  RotationSequenceAnglesUnits=deg  RotationMatrix=[1 0 0;0 1 0;0 0 1]  Quaternion=[1 0 0 0]  TranslationMethod=Cartesian  TranslationCartesianOffset=[-0.05 0 -0.06]  TranslationCartesianOffsetUnits=m  TranslationStandardAxis=+Z  TranslationStandardOffset=0  TranslationStandardOffsetUnits=m  TranslationROffset=0  TranslationROffsetUnits=m  TranslationThetaOffset=0  TranslationThetaOffsetUnits=deg  TranslationZOffset=0  TranslationZOffsetUnits=m
  RT_C_AXIS : sm_lib/Frames and Transforms/Rigid Transform  RotationMethod=StandardAxis  FollAlignAxisA=+X  BaseAlignAxisA=+Y  FollAlignAxisB=+Y  BaseAlignAxisB=+Z  RotationStandardAxis=+X  RotationAngle=-90  RotationAngleUnits=deg  RotationArbitraryAxis=[0 0 1]  RotationSequenceAxes=FollowerAxes  RotationSequence=XYX  RotationSequenceAngles=[0 0 0]  RotationSequenceAnglesUnits=deg  RotationMatrix=[1 0 0;0 1 0;0 0 1]  Quaternion=[1 0 0 0]  TranslationMethod=None  TranslationCartesianOffset=[0 0 0]  TranslationCartesianOffsetUnits=m  TranslationStandardAxis=+Z  TranslationStandardOffset=0  TranslationStandardOffsetUnits=m  TranslationROffset=0  TranslationROffsetUnits=m  TranslationThetaOffset=0  TranslationThetaOffsetUnits=deg  TranslationZOffset=0  TranslationZOffsetUnits=m
  RT_FORK : sm_lib/Frames and Transforms/Rigid Transform  RotationMethod=None  FollAlignAxisA=+X  BaseAlignAxisA=+Y  FollAlignAxisB=+Y  BaseAlignAxisB=+Z  RotationStandardAxis=+Z  RotationAngle=0  RotationAngleUnits=deg  RotationArbitraryAxis=[0 0 1]  RotationSequenceAxes=FollowerAxes  RotationSequence=XYX  RotationSequenceAngles=[0 0 0]  RotationSequenceAnglesUnits=deg  RotationMatrix=[1 0 0;0 1 0;0 0 1]  Quaternion=[1 0 0 0]  TranslationMethod=Cartesian  TranslationCartesianOffset=[-0.025 0 -0.03]  TranslationCartesianOffsetUnits=m  TranslationStandardAxis=+Z  TranslationStandardOffset=0  TranslationStandardOffsetUnits=m  TranslationROffset=0  TranslationROffsetUnits=m  TranslationThetaOffset=0  TranslationThetaOffsetUnits=deg  TranslationZOffset=0  TranslationZOffsetUnits=m
  RT_H : sm_lib/Frames and Transforms/Rigid Transform  RotationMethod=None  FollAlignAxisA=+X  BaseAlignAxisA=+Y  FollAlignAxisB=+Y  BaseAlignAxisB=+Z  RotationStandardAxis=+Z  RotationAngle=0  RotationAngleUnits=deg  RotationArbitraryAxis=[0 0 1]  RotationSequenceAxes=FollowerAxes  RotationSequence=XYX  RotationSequenceAngles=[0 0 0]  RotationSequenceAnglesUnits=deg  RotationMatrix=[1 0 0;0 1 0;0 0 1]  Quaternion=[1 0 0 0]  TranslationMethod=Cartesian  TranslationCartesianOffset=[-0.18 0 0.10]  TranslationCartesianOffsetUnits=m  TranslationStandardAxis=+Z  TranslationStandardOffset=0  TranslationStandardOffsetUnits=m  TranslationROffset=0  TranslationROffsetUnits=m  TranslationThetaOffset=0  TranslationThetaOffsetUnits=deg  TranslationZOffset=0  TranslationZOffsetUnits=m
  "RT_MOUNT_VIS " : sm_lib/Frames and Transforms/Rigid Transform  RotationMethod=None  FollAlignAxisA=+X  BaseAlignAxisA=+Y  FollAlignAxisB=+Y  BaseAlignAxisB=+Z  RotationStandardAxis=+Z  RotationAngle=0  RotationAngleUnits=deg  RotationArbitraryAxis=[0 0 1]  RotationSequenceAxes=FollowerAxes  RotationSequence=XYX  RotationSequenceAngles=[0 0 0]  RotationSequenceAnglesUnits=deg  RotationMatrix=[1 0 0;0 1 0;0 0 1]  Quaternion=[1 0 0 0]  TranslationMethod=Cartesian  TranslationCartesianOffset=[0 0 -0.02063]  TranslationCartesianOffsetUnits=m  TranslationStandardAxis=+Z  TranslationStandardOffset=0  TranslationStandardOffsetUnits=m  TranslationROffset=0  TranslationROffsetUnits=m  TranslationThetaOffset=0  TranslationThetaOffsetUnits=deg  TranslationZOffset=0  TranslationZOffsetUnits=m
  SWIVEL_SPEED : Scope
      settings: ActiveDisplayYMinimum=-0.099459675852848983  ActiveDisplayYMaximum=0.62076406504949133  DataLoggingMaxPoints=2000  DataLoggingVariableName=ScopeData3
  WHEEL_GEOMETRY : PMIOPort  Side=Right
  CHASSIS_FRAME : PMIOPort  Port=2  Side=Left
  wires:
  PS-Simulink Converter2/1 -> CASTER_ANGLE/1, EXPORT_caster_angle/1
  PS-Simulink Converter3/1 -> SWIVEL_SPEED/1, EXPORT_swivel_speed/1
  PS-Simulink Converter5/1 -> CASTER_WHEEL_SPEED/1, EXPORT_caster_roll_speed/1
  connections:
  RT_C/RConn1 -- RT_C_AXIS/LConn1
  RT_FORK/RConn1 -- FORK/RConn1
  CHASSIS_FRAME/RConn1 -- RT_H/LConn1
  RT_H/RConn1 -- "RT_MOUNT_VIS "/LConn1 -- J_SWIVEL/LConn1
  "RT_MOUNT_VIS "/RConn1 -- MOUNT_PLATE_VIS/RConn1
  FORK_VISUALS/LConn1 -- RT_FORK/LConn1 -- J_SWIVEL/RConn1 -- RT_C/LConn1
  J_SWIVEL/RConn3 -- PS-Simulink Converter3/LConn1
  J_SWIVEL/RConn2 -- PS-Simulink Converter2/LConn1
  RT_C_AXIS/RConn1 -- C_ROLL_JOINT/LConn1 -- CASTER_AXLE_VIS/RConn1
  WHEEL_GEOMETRY/RConn1 -- C_WHEEL/LConn1
  C_ROLL_JOINT/RConn1 -- C_WHEEL/RConn1
  C_ROLL_JOINT/RConn2 -- PS-Simulink Converter5/LConn1

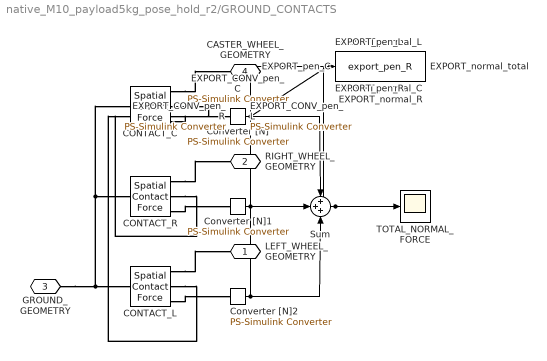
== system native_M10_payload5kg_pose_hold_r2/GROUND_CONTACTS ==
  " Converter [N]" : nesl_utility/PS-Simulink Converter  PhysicalDomain=network_engine_domain  SubClassName=ps_output  LeftPortType=input  RightPortType=output  PseudoPeriodic=off  Frequencies=[]  VectorFormat=inherit  Unit=N  AffineConversion=off
  " Converter [N]1" : nesl_utility/PS-Simulink Converter  PhysicalDomain=network_engine_domain  SubClassName=ps_output  LeftPortType=input  RightPortType=output  PseudoPeriodic=off  Frequencies=[]  VectorFormat=inherit  Unit=N  AffineConversion=off
  " Converter [N]2" : nesl_utility/PS-Simulink Converter  PhysicalDomain=network_engine_domain  SubClassName=ps_output  LeftPortType=input  RightPortType=output  PseudoPeriodic=off  Frequencies=[]  VectorFormat=inherit  Unit=N  AffineConversion=off
  CONTACT_C : sm_lib/Forces and Torques/Spatial Contact Force  SenseSeparationDistance=off  NormalForceType=SmoothSpringDamper  NormalStiffness=1e5  NormalStiffnessUnits=N/m  NormalDamping=500  NormalDampingUnits=N/(m/s)  NormalTransitionRegionWidth=1e-4  NormalTransitionRegionWidthUnits=m  FrictionType=SmoothStickSlip  CoefficientOfStaticFriction=0.5  CoefficientOfDynamicFriction=0.3  FrictionalCriticalVelocity=0.01  FrictionalCriticalVelocityUnits=m/s  SenseContactSignal=off  SensePenetrationDepth=on  SenseNormalVelocity=off  SenseTangentialVelocity=off  SensingForceTorqueDirection=BaseOnFollower  SensingForceTorqueResolutionFrame=ContactFrame  SenseNormalForce=on  SenseNormalForceMagnitude=off  SenseNormalTorque=off  SenseFrictionalForce=off  SenseFrictionalForceMagnitude=off  SenseFrictionalTorque=off  SenseTotalForce=off  SenseTotalTorque=off  SenseContactBaseRotation=off  SenseContactBaseTranslation=off  SenseContactFollowerRotation=off  SenseContactFollowerTranslation=off  ZeroCrossDetectContactStartAndEnd=off
  CONTACT_L : sm_lib/Forces and Torques/Spatial Contact Force  SenseSeparationDistance=off  NormalForceType=SmoothSpringDamper  NormalStiffness=1e5  NormalStiffnessUnits=N/m  NormalDamping=500  NormalDampingUnits=N/(m/s)  NormalTransitionRegionWidth=1e-4  NormalTransitionRegionWidthUnits=m  FrictionType=SmoothStickSlip  CoefficientOfStaticFriction=0.5  CoefficientOfDynamicFriction=0.3  FrictionalCriticalVelocity=0.01  FrictionalCriticalVelocityUnits=m/s  SenseContactSignal=off  SensePenetrationDepth=on  SenseNormalVelocity=off  SenseTangentialVelocity=off  SensingForceTorqueDirection=BaseOnFollower  SensingForceTorqueResolutionFrame=ContactFrame  SenseNormalForce=on  SenseNormalForceMagnitude=off  SenseNormalTorque=off  SenseFrictionalForce=off  SenseFrictionalForceMagnitude=off  SenseFrictionalTorque=off  SenseTotalForce=off  SenseTotalTorque=off  SenseContactBaseRotation=off  SenseContactBaseTranslation=off  SenseContactFollowerRotation=off  SenseContactFollowerTranslation=off  ZeroCrossDetectContactStartAndEnd=off
  CONTACT_R : sm_lib/Forces and Torques/Spatial Contact Force  SenseSeparationDistance=off  NormalForceType=SmoothSpringDamper  NormalStiffness=1e5  NormalStiffnessUnits=N/m  NormalDamping=500  NormalDampingUnits=N/(m/s)  NormalTransitionRegionWidth=1e-4  NormalTransitionRegionWidthUnits=m  FrictionType=SmoothStickSlip  CoefficientOfStaticFriction=0.5  CoefficientOfDynamicFriction=0.3  FrictionalCriticalVelocity=0.01  FrictionalCriticalVelocityUnits=m/s  SenseContactSignal=off  SensePenetrationDepth=on  SenseNormalVelocity=off  SenseTangentialVelocity=off  SensingForceTorqueDirection=BaseOnFollower  SensingForceTorqueResolutionFrame=ContactFrame  SenseNormalForce=on  SenseNormalForceMagnitude=off  SenseNormalTorque=off  SenseFrictionalForce=off  SenseFrictionalForceMagnitude=off  SenseFrictionalTorque=off  SenseTotalForce=off  SenseTotalTorque=off  SenseContactBaseRotation=off  SenseContactBaseTranslation=off  SenseContactFollowerRotation=off  SenseContactFollowerTranslation=off  ZeroCrossDetectContactStartAndEnd=off
  EXPORT_CONV_pen_C : nesl_utility/PS-Simulink Converter  PhysicalDomain=network_engine_domain  SubClassName=ps_output  LeftPortType=input  RightPortType=output  PseudoPeriodic=off  Frequencies=[]  VectorFormat=inherit  Unit=m  AffineConversion=off
  EXPORT_CONV_pen_L : nesl_utility/PS-Simulink Converter  PhysicalDomain=network_engine_domain  SubClassName=ps_output  LeftPortType=input  RightPortType=output  PseudoPeriodic=off  Frequencies=[]  VectorFormat=inherit  Unit=m  AffineConversion=off
  EXPORT_CONV_pen_R : nesl_utility/PS-Simulink Converter  PhysicalDomain=network_engine_domain  SubClassName=ps_output  LeftPortType=input  RightPortType=output  PseudoPeriodic=off  Frequencies=[]  VectorFormat=inherit  Unit=m  AffineConversion=off
  EXPORT_normal_C : ToWorkspace  VariableName=export_normal_C  SaveFormat=Timeseries  SampleTime=0.001
  EXPORT_normal_L : ToWorkspace  VariableName=export_normal_L  SaveFormat=Timeseries  SampleTime=0.001
  EXPORT_normal_R : ToWorkspace  VariableName=export_normal_R  SaveFormat=Timeseries  SampleTime=0.001
  EXPORT_normal_total : ToWorkspace  VariableName=export_normal_total  SaveFormat=Timeseries  SampleTime=0.001
  EXPORT_pen_C : ToWorkspace  VariableName=export_pen_C  SaveFormat=Timeseries  SampleTime=0.001
  EXPORT_pen_L : ToWorkspace  VariableName=export_pen_L  SaveFormat=Timeseries  SampleTime=0.001
  EXPORT_pen_R : ToWorkspace  VariableName=export_pen_R  SaveFormat=Timeseries  SampleTime=0.001
  Sum : Sum  Inputs=+++
  TOTAL_NORMAL_FORCE : Scope
      settings: ActiveDisplayYMinimum=-156359.16388109137  ActiveDisplayYMaximum=131206.96423001884  DataLoggingMaxPoints=2000  DataLoggingVariableName=ScopeData5
  LEFT_WHEEL_GEOMETRY : PMIOPort  Side=Left
  RIGHT_WHEEL_GEOMETRY : PMIOPort  Port=2  Side=Left
  GROUND_GEOMETRY : PMIOPort  Port=3  Side=Left
  CASTER_WHEEL_GEOMETRY : PMIOPort  Port=4  Side=Left
  wires:
  " Converter [N]"/1 -> Sum/1, EXPORT_normal_C/1
  " Converter [N]1"/1 -> Sum/2, EXPORT_normal_R/1
  " Converter [N]2"/1 -> Sum/3, EXPORT_normal_L/1
  Sum/1 -> TOTAL_NORMAL_FORCE/1, EXPORT_normal_total/1
  EXPORT_CONV_pen_L/1 -> EXPORT_pen_L/1
  EXPORT_CONV_pen_R/1 -> EXPORT_pen_R/1
  EXPORT_CONV_pen_C/1 -> EXPORT_pen_C/1
  connections:
  GROUND_GEOMETRY/RConn1 -- CONTACT_R/LConn1 -- CONTACT_C/LConn1 -- CONTACT_L/LConn1
  CONTACT_C/RConn3 -- " Converter [N]"/LConn1
  CONTACT_L/RConn3 -- " Converter [N]2"/LConn1
  CONTACT_C/RConn1 -- CASTER_WHEEL_GEOMETRY/RConn1
  CONTACT_L/RConn1 -- LEFT_WHEEL_GEOMETRY/RConn1
  CONTACT_R/RConn3 -- " Converter [N]1"/LConn1
  CONTACT_R/RConn1 -- RIGHT_WHEEL_GEOMETRY/RConn1
  CONTACT_L/RConn2 -- EXPORT_CONV_pen_L/LConn1
  CONTACT_R/RConn2 -- EXPORT_CONV_pen_R/LConn1
  CONTACT_C/RConn2 -- EXPORT_CONV_pen_C/LConn1

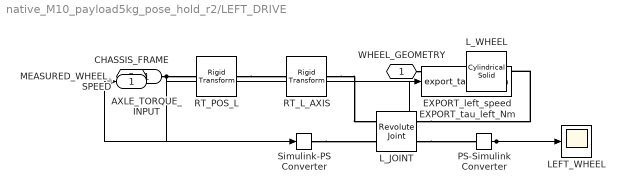
== system native_M10_payload5kg_pose_hold_r2/LEFT_DRIVE ==
  AXLE_TORQUE_INPUT : Inport
  EXPORT_left_speed : ToWorkspace  VariableName=export_left_speed  SaveFormat=Timeseries  SampleTime=0.001
  EXPORT_tau_left_Nm : ToWorkspace  VariableName=export_tau_left_Nm  SaveFormat=Timeseries  SampleTime=0.001
  LEFT_WHEEL : Scope
      settings: ActiveDisplayYMinimum=0.31488782970237528  ActiveDisplayYMaximum=2.1431155514621123  DataLoggingMaxPoints=2000
  L_JOINT : sm_lib/Joints/Revolute Joint  JointMode=Normal  CompositeWrenchDir=FollowerOnBase  CompositeWrenchFrame=BaseFrame  SenseConstraintForce=off  SenseConstraintTorque=off  SenseTotalForce=off  SenseTotalTorque=off  PositionTargetSpecify=off  PositionTargetPriority=High  PositionTargetValue=0  PositionTargetValueUnits=deg  VelocityTargetSpecify=off  VelocityTargetPriority=High  VelocityTargetValue=0  VelocityTargetValueUnits=deg/s  EquilibriumPosition=0  EquilibriumPositionUnits=deg  SpringStiffness=0  SpringStiffnessUnits=N*m/deg  DampingCoefficient=0  DampingCoefficientUnits=N*m/(deg/s)  LowerLimitSpecify=off  LowerLimitBound=-90  LowerLimitBoundUnits=deg  LowerLimitStiffness=1e4  LowerLimitStiffnessUnits=N*m/deg  LowerLimitDamping=10  LowerLimitDampingUnits=N*m/(deg/s)  LowerLimitTransitionRegionWidth=0.1  LowerLimitTransitionRegionWidthUnits=deg  UpperLimitSpecify=off  UpperLimitBound=90  UpperLimitBoundUnits=deg  UpperLimitStiffness=1e4  UpperLimitStiffnessUnits=N*m/deg  UpperLimitDamping=10  UpperLimitDampingUnits=N*m/(deg/s)  UpperLimitTransitionRegionWidth=0.1  UpperLimitTransitionRegionWidthUnits=deg  TorqueActuationMode=InputTorque  MotionActuationMode=ComputedMotion  SensePosition=off  SenseVelocity=on  SenseAcceleration=off  SenseTorqueForce=off  SenseLowerLimitTorqueForce=off  SenseUpperLimitTorqueForce=off
  L_WHEEL : sm_lib/Body Elements/Cylindrical Solid  CylinderRadius=0.075  CylinderRadiusUnits=m  CylinderLength=0.03  CylinderLengthUnits=m  ExportEntireGeometry=on  InertiaType=CalculateFromGeometry  BasedOnType=Mass  Density=1000  DensityUnits=kg/m^3  Mass=0.4  MassUnits=kg  CenterOfMass=[0 0 0]  CenterOfMassUnits=m  MomentsOfInertia=[1 1 1]  MomentsOfInertiaUnits=kg*m^2  ProductsOfInertia=[0 0 0]  ProductsOfInertiaUnits=kg*m^2  GraphicType=FromGeometry  MarkerShape=Sphere  MarkerSize=10  GraphicVisPropType=SimpleVisualProperties  GraphicDiffuseColor=[0.5 0.5 0.5]  GraphicOpacity=1  GraphicSpecularColor=[0.5 0.5 0.5 1.0]  GraphicAmbientColor=[0.15 0.15 0.15 1.0]  GraphicEmissiveColor=[0.0 0.0 0.0 1.0]  GraphicShininess=75  DoExposeReferenceFrame=on  SerializedFrames=<Frames/>
  PS-Simulink Converter : nesl_utility/PS-Simulink Converter  PhysicalDomain=network_engine_domain  SubClassName=ps_output  LeftPortType=input  RightPortType=output  PseudoPeriodic=off  Frequencies=[]  VectorFormat=inherit  Unit=rad/s  AffineConversion=off
  RT_L_AXIS : sm_lib/Frames and Transforms/Rigid Transform  RotationMethod=StandardAxis  FollAlignAxisA=+X  BaseAlignAxisA=+Y  FollAlignAxisB=+Y  BaseAlignAxisB=+Z  RotationStandardAxis=+X  RotationAngle=-90  RotationAngleUnits=deg  RotationArbitraryAxis=[0 0 1]  RotationSequenceAxes=FollowerAxes  RotationSequence=XYX  RotationSequenceAngles=[0 0 0]  RotationSequenceAnglesUnits=deg  RotationMatrix=[1 0 0;0 1 0;0 0 1]  Quaternion=[1 0 0 0]  TranslationMethod=None  TranslationCartesianOffset=[0 0 0]  TranslationCartesianOffsetUnits=m  TranslationStandardAxis=+Z  TranslationStandardOffset=0  TranslationStandardOffsetUnits=m  TranslationROffset=0  TranslationROffsetUnits=m  TranslationThetaOffset=0  TranslationThetaOffsetUnits=deg  TranslationZOffset=0  TranslationZOffsetUnits=m
  RT_POS_L : sm_lib/Frames and Transforms/Rigid Transform  RotationMethod=None  FollAlignAxisA=+X  BaseAlignAxisA=+Y  FollAlignAxisB=+Y  BaseAlignAxisB=+Z  RotationStandardAxis=+Z  RotationAngle=0  RotationAngleUnits=deg  RotationArbitraryAxis=[0 0 1]  RotationSequenceAxes=FollowerAxes  RotationSequence=XYX  RotationSequenceAngles=[0 0 0]  RotationSequenceAnglesUnits=deg  RotationMatrix=[1 0 0;0 1 0;0 0 1]  Quaternion=[1 0 0 0]  TranslationMethod=Cartesian  TranslationCartesianOffset=[0 0.19 0.075]  TranslationCartesianOffsetUnits=m  TranslationStandardAxis=+Z  TranslationStandardOffset=0  TranslationStandardOffsetUnits=m  TranslationROffset=0  TranslationROffsetUnits=m  TranslationThetaOffset=0  TranslationThetaOffsetUnits=deg  TranslationZOffset=0  TranslationZOffsetUnits=m
  Simulink-PS Converter : nesl_utility/Simulink-PS Converter  PhysicalDomain=network_engine_domain  SubClassName=ps_input  LeftPortType=input  RightPortType=output  PseudoPeriodic=off  Frequencies=[]  NoiseDistribution=none  NoiseParameters=[]  Unit=N*m  AffineConversion=off  FilteringAndDerivatives=zero  SimscapeFilterOrder=1  InputFilterTimeConstant=0.001  UdotUserProvided=0
  WHEEL_GEOMETRY : PMIOPort  Side=Right
  CHASSIS_FRAME : PMIOPort  Port=2  Side=Left
  MEASURED_WHEEL_SPEED : Outport
  wires:
  PS-Simulink Converter/1 -> LEFT_WHEEL/1, EXPORT_left_speed/1, MEASURED_WHEEL_SPEED/1
  AXLE_TORQUE_INPUT/1 -> Simulink-PS Converter/1, EXPORT_tau_left_Nm/1
  connections:
  WHEEL_GEOMETRY/RConn1 -- L_WHEEL/LConn1
  RT_L_AXIS/RConn1 -- L_JOINT/LConn1
  CHASSIS_FRAME/RConn1 -- RT_POS_L/LConn1
  RT_POS_L/RConn1 -- RT_L_AXIS/LConn1
  Simulink-PS Converter/RConn1 -- L_JOINT/LConn2
  L_JOINT/RConn2 -- PS-Simulink Converter/LConn1
  L_JOINT/RConn1 -- L_WHEEL/RConn1
